simulink model "OSWEC_RO"  (R2023b)
settings: Solver=ode4  StartTime=0  StopTime=300  FixedStep=0.01  MaxStep=0.01  RelTol=1e-3  AbsTol=1e-3  EnableMultiTasking=on
values from neighbouring files (symbols this model uses):
  inertiaBlock = 1e-3    (= 0.001)    [wecSimInputFile.m]
  simu = simulationClass()    [wecSimInputFile.m]
undefined symbols (not defined in the file or in its folder): body, constraint, pto
libraries: fl_lib x17, nesl_utility x11, sh_lib x10, WECSim_Lib_Constraints x4, WECSim_Lib_Body_Elements x2, WECSim_Lib_Frames x1, sm_lib x1, fl_ps_legacy_lib x1, WECSim_Lib_PTOs x1
settings Model: Creator=mlawson  LastModifiedBy=jtgrasb
settings SolverCC: AutoScaleAbsTol=off  ZeroCrossControl=DisableAll  AlgebraicLoopSolver=TrustRegion  AutoInsertRateTranBlk=on
settings DataIOCC: SaveFormat=Array  SaveOutput=off  SaveTime=off  ReturnWorkspaceOutputs=off
settings OptimizationCC: LifeSpan=inf  SimCompilerOptimization=on
settings DebuggingCC: MergeDetectMultiDrivingBlocksExec=none  SolverPrmCheckMsg=warning  UnconnectedInputMsg=warning  UnconnectedOutputMsg=warning  UnconnectedLineMsg=warning  AllowSymbolicDim=off  StateNameClashWarn=warning  SFUnexpectedBacktrackingDiag=warning  SFNoUnconditionalDefaultTransitionDiag=warning  SFExecutionAtInitializationDiag=none  ArithmeticOperatorsInVariantConditions=warning
settings HardwareCC: ProdBitPerPointer=32  ProdBitPerSizeT=32  ProdBitPerPtrDiffT=32  ProdLargestAtomicFloat=None  ProdIntDivRoundTo=Undefined  ProdEndianess=Unspecified  ProdWordSize=32  ProdHWDeviceType=32-bit Generic
settings ModelReferenceCC: EnableRefExpFcnMdlSchedulingChecks=on  PropagateSignalLabelsOutOfModel=off
settings SFSimCC: SimUseLocalCustomCode=off  CustomCodeUndefinedFunction=UseInterfaceOnly
settings RTWCC: RTWUseLocalCustomCode=off  DLArmComputeVersion=19.05
settings CodeAppCC: StateflowObjectComments=on
settings GRTTargetCC: TargetLangStandard=C89/C90 (ANSI)
settings ConfigComp: CovMetricSettings=dw  CovSaveCumulativeToWorkspaceVar=on  CovSaveSingleToWorkspaceVar=on  CovExternalEMLEnable=off  CovSFcnEnable=off
settings SimscapeCC: SimscapeNormalizeSystem=off  SimscapeLogType=all  SimscapeLogLimitData=off  SimscapeLogDataHistory=100000
settings ConfigurationSet: Description=SimMechanics 2G
settings ExplorerConfigSet: SimMechanicsOpenEditorOnUpdate=off  InternalSimMechanicsExplorerSettings="<ExplorerConfiguration><canonicalview>default</canonicalview><TilePanel><TileInfo><Tiles Columns=\"1\" Count=\"1\" Rows=\"1\"><Column Left=\"2\" Weight=\"1\"/><Column Left=\"1335\"/><Row Top=\"2\" Weight=\"1\"/><Row Top=\"911\"/><Tile Height=\"1\" Width=\"1\" X=\"0\" Y=\"0\"/></Tiles></TileInfo><SceneInfo><SceneViewer><BGColor><R>0.60000002384185791</R><G>0.60000002384185791</G><B>0.60000002384185791</B></BGColor><Camera><Position><X>365.37645888990272</X><Y>-369.82486814446582</Y><Z>359.64809521743916</Z></Position><Center><X>-6.7351450971904585</X><Y>2.2867358426280204</Y><Z>-12.463508769654169</Z></Center><Up><X>-0.40824829046386307</X><Y>0.40824829046386307</Y><Z>0.81649658092772615</Z></Up><Left>-57.820127362122818</Left><Right>57.820127362122818</Right><Bottom>-38.308817187253304</Bottom><Top>38.308817187253304</Top></Camera></SceneViewer></SceneInfo></TilePanel></ExplorerConfiguration>"

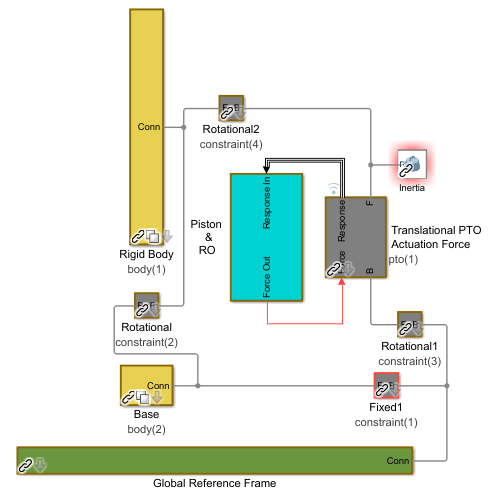
[thumbnail: Simulink's stored preview of the top-level diagram]
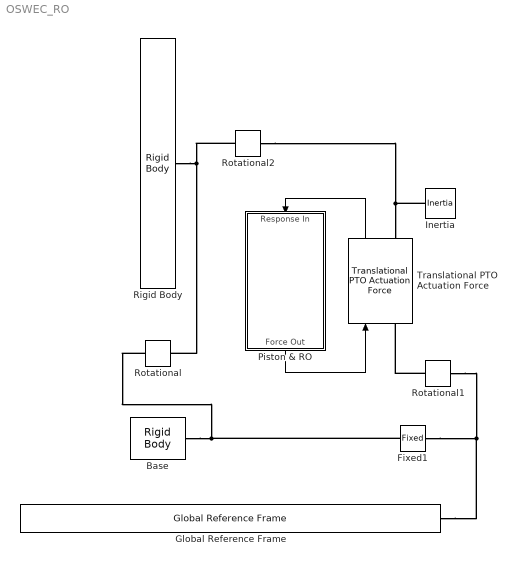
== system OSWEC_RO ==
  Base : WECSim_Lib_Body_Elements/Rigid Body  body=body(2)
  Fixed1 : WECSim_Lib_Constraints/Fixed  constraint=constraint(1)
      settings: AttributesFormatString=%<constraint>
  Global Reference Frame : WECSim_Lib_Frames/Global Reference Frame  waves=waves  simu=simu
  Inertia : sm_lib/Body Elements/Inertia  InertiaType=PointMass  Mass=inertiaBlock  MassUnits=kg  CenterOfMass=[0 0 0]  CenterOfMassUnits=m  MomentsOfInertia=[1 1 1]  MomentsOfInertiaUnits=kg*m^2  ProductsOfInertia=[1 1 1]  ProductsOfInertiaUnits=kg*m^2  GraphicType=Marker  MarkerShape=Inertia  MarkerSize=20  GraphicVisPropType=SimpleVisualProperties  GraphicDiffuseColor=[0.5 0.5 0.5]  GraphicSpecularColor=[0.5 0.5 0.5 1.0]  GraphicAmbientColor=[0.15 0.15 0.15 1.0]  GraphicEmissiveColor=[0.0 0.0 0.0 1.0]  GraphicShininess=75  GraphicOpacity=1.0
  "Piston & RO   " : Subsystem
  Rigid Body : WECSim_Lib_Body_Elements/Rigid Body  body=body(1)
  Rotational : WECSim_Lib_Constraints/Rotational  constraint=constraint(2)
      settings: AttributesFormatString=%<constraint>
  Rotational1 : WECSim_Lib_Constraints/Rotational  constraint=constraint(3)
      settings: AttributesFormatString=%<constraint>
  Rotational2 : WECSim_Lib_Constraints/Rotational  constraint=constraint(4)
      settings: AttributesFormatString=%<constraint>
  Translational PTO Actuation Force : WECSim_Lib_PTOs/Translational PTO Actuation Force  pto=pto(1)
      settings: AttributesFormatString=%<pto>
  wires:
  "Piston & RO   "/1(Force Out) -> Translational PTO Actuation Force/1
  Translational PTO Actuation Force/1 -> "Piston & RO   "/1(Response In)
  connections:
  Fixed1/LConn1 -- Global Reference Frame/RConn1 -- Rotational1/LConn1
  Fixed1/RConn1 -- Rotational/LConn1 -- Base/RConn1
  Rotational2/RConn1 -- Rigid Body/RConn1 -- Rotational/RConn1
  Rotational1/RConn1 -- Translational PTO Actuation Force/LConn1
  Rotational2/LConn1 -- Inertia/RConn1 -- Translational PTO Actuation Force/RConn1

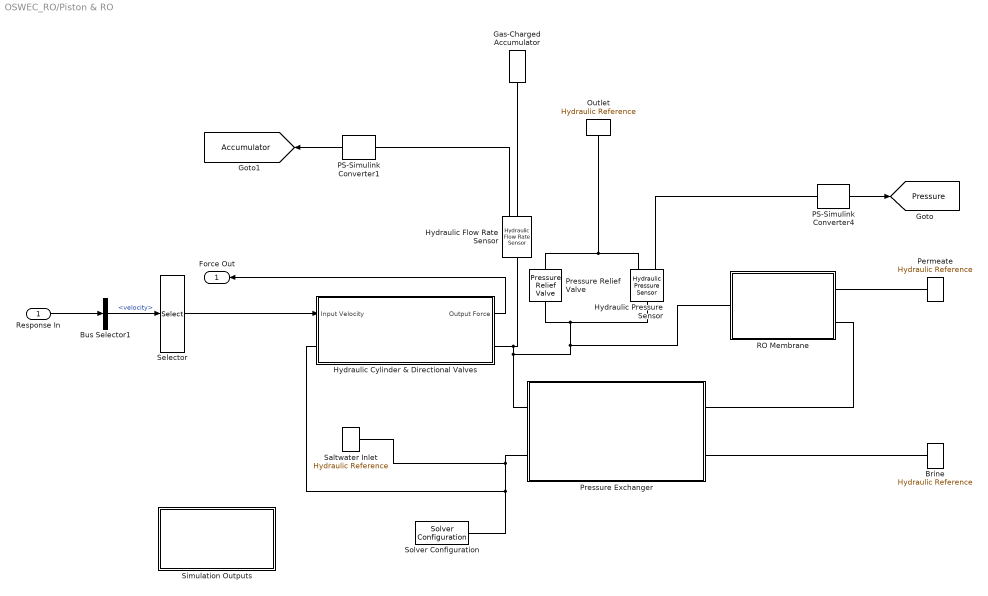
== system OSWEC_RO/Piston & RO    ==
  Response In : Inport
  "Brine " : fl_lib/Hydraulic/Hydraulic Elements/Hydraulic Reference
  Bus Selector1 : BusSelector  OutputSignals=velocity
  Gas-Charged Accumulator : sh_lib/Accumulators/Gas-Charged Accumulator  capacity=4 m^3  dead_volume=4e-5 m^3  pr_preload=30e5 Pa  k_sh=1.4  stiff_coeff=1e7 Pa/m^3  penetr_coeff=1e7 s*Pa/m^6  flow_rate_specify=off  flow_rate_priority=None  flow_rate=0 m^3/s  flow_rate_nominal_specify=off  flow_rate_nominal_unit=m^3/s  flow_rate_nominal_value=1  liquid_volume_specify=on  liquid_volume_priority=High  liquid_volume=0 m^3  liquid_volume_nominal_specify=off  liquid_volume_nominal_unit=m^3  liquid_volume_nominal_value=1  liquid_pressure_specify=off  liquid_pressure_priority=None  liquid_pressure=1.01325e+5 Pa  liquid_pressure_nominal_specify=off  liquid_pressure_nominal_unit=Pa  liquid_pressure_nominal_value=1
      settings: InternalSimscapePortConfiguration="{\"Bottom\":[],\"Left\":[],\"Right\":[{\"id\":\"A\",\"label\":\"A\",\"type\":\"foundation.hydraulic.hydraulic\"}],\"Top\":[]}"
  Hydraulic Flow Rate Sensor : fl_lib/Hydraulic/Hydraulic Sensors/Hydraulic Flow Rate Sensor
  Hydraulic Cylinder & Directional Valves : Subsystem
      mask Display: image('Images/HydraulicCylinder.png');
  Hydraulic Pressure Sensor : fl_lib/Hydraulic/Hydraulic Sensors/Hydraulic Pressure Sensor
  Outlet : fl_lib/Hydraulic/Hydraulic Elements/Hydraulic Reference
  PS-Simulink Converter1 : nesl_utility/PS-Simulink Converter  PhysicalDomain=network_engine_domain  SubClassName=ps_output  LeftPortType=input  RightPortType=output  PseudoPeriodic=off  Frequencies=[]  VectorFormat=1-D array  Unit=1  AffineConversion=off
  PS-Simulink Converter4 : nesl_utility/PS-Simulink Converter  PhysicalDomain=network_engine_domain  SubClassName=ps_output  LeftPortType=input  RightPortType=output  PseudoPeriodic=off  Frequencies=[]  VectorFormat=1-D array  Unit=1  AffineConversion=off
  Permeate : fl_lib/Hydraulic/Hydraulic Elements/Hydraulic Reference
  Pressure Relief Valve : sh_lib/Valves/Pressure Control Valves/Pressure Relief Valve  valve_area_spec=1  p_diff_TLU=[30.15e5 : 15e3 : 31.35e5] Pa  area_TLU=[1 : 1 : 9] .* 1e-5 m^2  area_max=2.67e-2 m^2  pres_set=56e5 Pa  reg_range=1e5 Pa  C_d=0.7  A_leak=1e-12 m^2  lam_spec=1  B_lam=0.999  Re_cr=12  dynamic=1  tau=0.1 s  area_init=1e-12 m^2
      settings: InternalSimscapePortConfiguration="{\"Bottom\":[],\"Left\":[{\"id\":\"A\",\"label\":\"A\",\"type\":\"foundation.hydraulic.hydraulic\"}],\"Right\":[{\"id\":\"B\",\"label\":\"B\",\"type\":\"foundation.hydraulic.hydraulic\"}],\"Top\":[]}"
  Pressure Exchanger : Subsystem
      mask Display: image('Images/PressureExchanger.png');
  RO Membrane : Subsystem
      mask Display: image('Images/ReverseOsmosisMembrane.jpg');
  Saltwater Inlet : fl_lib/Hydraulic/Hydraulic Elements/Hydraulic Reference
  Selector : Selector  InputPortWidth=6  IndexOptions=Index vector (dialog)  Indices=3  OutputSizes=1
  Simulation Outputs : Subsystem
  Solver Configuration : nesl_utility/Solver Configuration  PhysicalDomain=network_engine_domain  SubClassName=solver  LeftPortType=input  RightPortType=generic  Tones=[]  Harmonics=[]  SimulateNoise=off  Profile=off  UseLocalSampling=off  EnableSwitchedLinearOptims=on  FrequencyDomain=off  UseCCode=off  RelTol=0.001  AbsTol=1e-06  MinStep=1e-09  ToWorkspace=off  RevertToSquareIcSolve=off  NumHomotopyIterations=100  PhasorMode=off  PhasorModeNumHarmonics=1  ConsistencySolver=NEWTON_FTOL  IndexReductionMethod=DerivativeReplacement  DoDC=on  ResidualTolerance=1e-09  ConsistencyTolSource=GLOBAL  ConsistencyAbsTol=0.001  ConsistencyRelTol=0.001  ConsistencyTolFactor=0.001  UseLocalSolver=on  LocalSolverChoice=NE_BACKWARD_EULER_ADVANCER  ResolveIndetEquations=on  FunctionEvalNumThread=1  LocalSolverSampleTime=simu.dt  DoFixedCost=on  MaxNonlinIter=3  MaxModeIter=2  ComputeImpulses=off  ImpulseIterations=2  LinearAlgebra=Sparse  LinearAlgebraNumThread=0  EquationFormulation=NE_TIME_EF  DelaysMemoryBudget=1024  AutomaticFiltering=on  FilteringTimeConstant=0.001  PartitionStorageMethod=AS_NEEDED  PartitionMemoryBudget=1024  PartitionMethod=FAST  MultibodyUseLocalSolver=off  MultibodyLocalSolverChoice=ODE1  MultibodyLocalSolverSampleTime=0.001
  Force Out : Outport  VectorParamsAs1DForOutWhenUnconnected=off
  tag scope: Accumulator=global, Pressure=global
  wires:
  Hydraulic Cylinder & Directional Valves/1(Output Force) -> Force Out/1
  PS-Simulink Converter4/1 -> [Pressure]
  PS-Simulink Converter1/1 -> [Accumulator]
  Response In/1 -> Bus Selector1/1
  Bus Selector1/1 -> Selector/1  "<velocity>"
  Selector/1 -> Hydraulic Cylinder & Directional Valves/1(Input Velocity)
  connections:
  Hydraulic Cylinder & Directional Valves/LConn1 -- Pressure Exchanger/LConn2 -- Saltwater Inlet/LConn1 -- Solver Configuration/RConn1
  Outlet/LConn1 -- Hydraulic Pressure Sensor/RConn1 -- Pressure Relief Valve/RConn1
  Permeate/LConn1 -- RO Membrane/RConn1
  PS-Simulink Converter4/LConn1 -- Hydraulic Pressure Sensor/RConn2
  RO Membrane/RConn2 -- Pressure Exchanger/RConn1
  "Brine "/LConn1 -- Pressure Exchanger/RConn2
  Hydraulic Flow Rate Sensor/RConn1 -- PS-Simulink Converter1/LConn1
  Hydraulic Cylinder & Directional Valves/RConn1 -- Hydraulic Flow Rate Sensor/LConn1 -- Pressure Exchanger/LConn1 -- Hydraulic Pressure Sensor/LConn1 -- Pressure Relief Valve/LConn1 -- RO Membrane/LConn1
  Hydraulic Flow Rate Sensor/RConn2 -- Gas-Charged Accumulator/RConn1

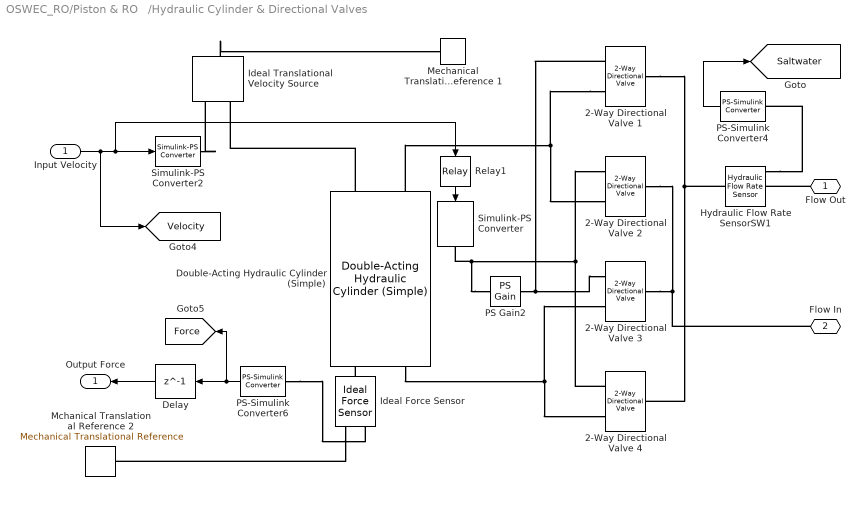
== system OSWEC_RO/Piston & RO   /Hydraulic Cylinder & Directional Valves ==
  Input Velocity : Inport
  2-Way Directional Valve {1..4} (4 alike) : sh_lib/Valves/Directional Valves/2-Way Directional Valve  mdl_type=1  area_max=5e-2 m^2  opening_max=1 m  opening_tab=[-0.002, 0.0, 0.002, 0.005, 0.015] m  area_tab=[1.0e-9, 2.0352e-7, 4.0736e-5, 0.00011438, 0.00034356] m^2  pressure_tab=[-10000000.0, -5000000.0, -2000000.0, 2000000.0, 5000000.0, 10000000.0] Pa  flow_rate_tab=[-1.0e-7, -7.0711e-8, -4.4721e-8, 4.4721e-8, 7.0711e-8, 1.0e-7; -2.0352e-5, -1.4391e-5, -9.1017e-6, 9.1017e-6, 1.4391e-5, 2.0352e-5; -0.0040736, -0.0028805, -0.0018218, 0.0018218, 0.0028805, 0.0040736; -0.011438, -0.0080879, -0.0051152, 0.0051152, 0.0080879, 0.011438; -0.034356, -0.024293, -0.015364, 0.015364, 0.024293, 0.034356] m^3/s  interp_method=1  extrap_method=1  C_d=0.7  x_0=0 m  A_leak=1e-8 m^2  lam_spec=1  B_lam=0.999  Re_cr=12
      settings: InternalSimscapePortConfiguration="{\"Bottom\":[],\"Left\":[{\"id\":\"S\",\"label\":\"S\",\"type\":\"input\"},{\"id\":\"A\",\"label\":\"A\",\"type\":\"foundation.hydraulic.hydraulic\"}],\"Right\":[{\"id\":\"B\",\"label\":\"B\",\"type\":\"foundation.hydraulic.hydraulic\"}],\"Top\":[]}"
  Delay : Delay  DelayLength=1  InitialCondition=0
  Double-Acting Hydraulic Cylinder (Simple) : sh_lib/Hydraulic Cylinders/Double-Acting Hydraulic Cylinder (Simple)  area_A=0.26 m^2  area_B=0.26 m^2  stroke=12 m  init_pos=6 m  penetr_coeff=1e12 s*N/m^2  or=1
      settings: InternalSimscapePortConfiguration="{\"Bottom\":[],\"Left\":[{\"id\":\"C\",\"label\":\"C\",\"type\":\"foundation.mechanical.translational.translational\"},{\"id\":\"A\",\"label\":\"A\",\"type\":\"foundation.hydraulic.hydraulic\"}],\"Right\":[{\"id\":\"R\",\"label\":\"R\",\"type\":\"foundation.mechanical.translational.translational\"},{\"id\":\"B\",\"label\":\"B\",\"type\":\"foundation.hydraulic.hydraulic\"}],\"Top\":[]}"
  Hydraulic Flow Rate SensorSW1 : fl_lib/Hydraulic/Hydraulic Sensors/Hydraulic Flow Rate Sensor
  Ideal Force Sensor : fl_lib/Mechanical/Mechanical Sensors/Ideal Force Sensor
  Ideal Translational Velocity Source : fl_lib/Mechanical/Mechanical Sources/Ideal Translational Velocity Source
  Mchanical Translational Reference 2 : fl_lib/Mechanical/Translational Elements/Mechanical Translational Reference
  Mechanical Translational Reference 1 : fl_lib/Mechanical/Translational Elements/Mechanical Translational Reference
  PS Gain2 : fl_ps_legacy_lib/Legacy Physical Signals/Functions/PS Gain  gain=-1
  PS-Simulink Converter4 : nesl_utility/PS-Simulink Converter  PhysicalDomain=network_engine_domain  SubClassName=ps_output  LeftPortType=input  RightPortType=output  PseudoPeriodic=off  Frequencies=[]  VectorFormat=1-D array  Unit=1  AffineConversion=off
  PS-Simulink Converter6 : nesl_utility/PS-Simulink Converter  PhysicalDomain=network_engine_domain  SubClassName=ps_output  LeftPortType=input  RightPortType=output  PseudoPeriodic=off  Frequencies=[]  VectorFormat=1-D array  Unit=1  AffineConversion=off
  Relay1 : Relay  OnSwitchValue=0  OffSwitchValue=0  OffOutputValue=-1  ZeroCross=off
  Simulink-PS Converter : nesl_utility/Simulink-PS Converter  PhysicalDomain=network_engine_domain  SubClassName=ps_input  LeftPortType=input  RightPortType=output  PseudoPeriodic=off  Frequencies=[]  NoiseDistribution=none  NoiseParameters=[]  Unit=1  AffineConversion=off  FilteringAndDerivatives=provide  SimscapeFilterOrder=2  InputFilterTimeConstant=0.01  UdotUserProvided=0
  Simulink-PS Converter2 : nesl_utility/Simulink-PS Converter  PhysicalDomain=network_engine_domain  SubClassName=ps_input  LeftPortType=input  RightPortType=output  PseudoPeriodic=off  Frequencies=[]  NoiseDistribution=none  NoiseParameters=[]  Unit=1  AffineConversion=off  FilteringAndDerivatives=provide  SimscapeFilterOrder=1  InputFilterTimeConstant=0.01  UdotUserProvided=0
  Flow Out : PMIOPort  Side=Right
  Flow In : PMIOPort  Port=2  Side=Left
  Output Force : Outport  VectorParamsAs1DForOutWhenUnconnected=off
  tag scope: Force=global, Saltwater=global, Velocity=global
  wires:
  Relay1/1 -> Simulink-PS Converter/1
  PS-Simulink Converter6/1 -> Delay/1, [Force]
  Input Velocity/1 -> [Velocity], Relay1/1, Simulink-PS Converter2/1
  Delay/1 -> Output Force/1
  PS-Simulink Converter4/1 -> [Saltwater]
  connections:
  2-Way Directional Valve 1/LConn2 -- Double-Acting Hydraulic Cylinder (Simple)/RConn2 -- 2-Way Directional Valve 2/LConn2
  2-Way Directional Valve 1/RConn1 -- Hydraulic Flow Rate SensorSW1/LConn1 -- 2-Way Directional Valve 4/RConn1
  2-Way Directional Valve 3/RConn1 -- Flow In/RConn1 -- 2-Way Directional Valve 2/RConn1
  2-Way Directional Valve 3/LConn1 -- 2-Way Directional Valve 1/LConn1 -- PS Gain2/RConn1
  Double-Acting Hydraulic Cylinder (Simple)/LConn2 -- 2-Way Directional Valve 3/LConn2 -- 2-Way Directional Valve 4/LConn2
  PS Gain2/LConn1 -- Simulink-PS Converter/RConn1 -- 2-Way Directional Valve 4/LConn1 -- 2-Way Directional Valve 2/LConn1
  Ideal Translational Velocity Source/LConn1 -- Mechanical Translational Reference 1/LConn1
  Simulink-PS Converter2/RConn1 -- Ideal Translational Velocity Source/RConn1
  PS-Simulink Converter6/LConn1 -- Ideal Force Sensor/RConn2
  Double-Acting Hydraulic Cylinder (Simple)/RConn1 -- Ideal Translational Velocity Source/RConn2
  Hydraulic Flow Rate SensorSW1/RConn1 -- PS-Simulink Converter4/LConn1
  Flow Out/RConn1 -- Hydraulic Flow Rate SensorSW1/RConn2
  Ideal Force Sensor/LConn1 -- Double-Acting Hydraulic Cylinder (Simple)/LConn1
  Ideal Force Sensor/RConn1 -- Mchanical Translational Reference 2/LConn1

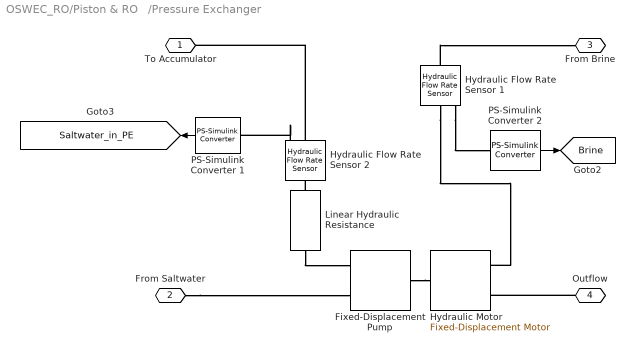
== system OSWEC_RO/Piston & RO   /Pressure Exchanger ==
  Fixed-Displacement Pump : sh_lib/Pumps and Motors/Fixed-Displacement Pump  D=(5e-6)*0.95 m^3/rad  loss_spec=1  w_nominal=188 rad/s  pr_nominal=100e5 Pa  visc_nominal=18 cSt  dens_nominal=900 kg/m^3  efficiency_vol=1  no_load_torque=0 N*m  torque_pressure_coeff=1*(5e-6)*((1)/(1)-1 ) N*m/Pa  p_diff_eff_TLU=[100000.0, 1000000.0, 2000000.0] Pa  omega_eff_TLU=[25.0, 50.0, 100.0, 200.0, 300.0, 400.0] rad/s  vol_eff_TLU=[0.816, 0.908, 0.954, 0.977, 0.981, 0.984; 0.325, 0.663, 0.831, 0.916, 0.925, 0.946; 0.137, 0.568, 0.78, 0.892, 0.893, 0.91]  mech_eff_TLU=[0.996, 0.996, 0.996, 0.996, 0.996, 0.996; 0.988, 0.989, 0.989, 0.989, 0.989, 0.99; 0.981, 0.981, 0.982, 0.982, 0.983, 0.984]  p_diff_loss_TLU=[100000.0, 1000000.0, 2000000.0] Pa  omega_loss_TLU=[25.0, 50.0, 100.0, 200.0, 300.0, 400.0] rad/s  vol_loss_TLU=[0.023, 0.023, 0.023, 0.023, 0.0285, 0.032; 0.0844, 0.0842, 0.0845, 0.084, 0.1125, 0.108; 0.1079, 0.108, 0.11, 0.108, 0.1605, 0.18] * 1e-3 m^3/s  mech_loss_TLU=[0.002, 0.002, 0.002, 0.002, 0.002, 0.002; 0.0607, 0.0556, 0.0556, 0.0556, 0.0556, 0.0505; 0.1937, 0.1937, 0.1833, 0.1833, 0.1729, 0.1626] N*m  pressure_threshold=1e5 Pa  omega_threshold=10 rad/s  quadrant_check=0  pressure_check=0  min_valid_pressure=0 Pa  vol_eff_min=1e-3  vol_eff_max=1  mech_eff_min=1e-3  mech_eff_max=1
      settings: InternalSimscapePortConfiguration="{\"Bottom\":[],\"Left\":[{\"id\":\"S\",\"label\":\"S\",\"type\":\"foundation.mechanical.rotational.rotational\"}],\"Right\":[{\"id\":\"P\",\"label\":\"P\",\"type\":\"foundation.hydraulic.hydraulic\"},{\"id\":\"T\",\"label\":\"T\",\"type\":\"foundation.hydraulic.hydraulic\"}],\"Top\":[]}"
  Hydraulic Motor : sh_lib/Pumps and Motors/Fixed-Displacement Motor  D=5e-6 m^3/rad  loss_spec=1  w_nominal=188 rad/s  pr_nominal=100e5 Pa  visc_nominal=18 cSt  dens_nominal=900 kg/m^3  efficiency_vol=1  no_load_torque=0 N*m  torque_pressure_coeff=1*(5e-6)*( 1-(1)/(1)) N*m/Pa  p_diff_eff_TLU=[100000.0, 1000000.0, 2000000.0] Pa  omega_eff_TLU=[25.0, 50.0, 100.0, 200.0, 300.0, 400.0] rad/s  vol_eff_TLU=[0.816, 0.908, 0.954, 0.977, 0.981, 0.984; 0.325, 0.663, 0.831, 0.916, 0.925, 0.946; 0.137, 0.568, 0.78, 0.892, 0.893, 0.91]  mech_eff_TLU=[0.996, 0.996, 0.996, 0.996, 0.996, 0.996; 0.988, 0.989, 0.989, 0.989, 0.989, 0.99; 0.981, 0.981, 0.982, 0.982, 0.983, 0.984]  p_diff_loss_TLU=[100000.0, 1000000.0, 2000000.0] Pa  omega_loss_TLU=[25.0, 50.0, 100.0, 200.0, 300.0, 400.0] rad/s  vol_loss_TLU=[0.0282, 0.0253, 0.0241, 0.0235, 0.0291, 0.0325; 0.2596, 0.1271, 0.1017, 0.0917, 0.1216, 0.1142; 0.7874, 0.1901, 0.141, 0.1211, 0.1797, 0.1978] * 1e-3 m^3/s  mech_loss_TLU=[0.002, 0.002, 0.002, 0.002, 0.002, 0.002; 0.06, 0.055, 0.055, 0.055, 0.055, 0.05; 0.19, 0.19, 0.18, 0.18, 0.17, 0.16] N*m  pressure_threshold=1e5 Pa  omega_threshold=10 rad/s  quadrant_check=0  pressure_check=0  min_valid_pressure=0 Pa  vol_eff_min=1e-3  vol_eff_max=1  mech_eff_min=1e-3  mech_eff_max=1
      settings: InternalSimscapePortConfiguration="{\"Bottom\":[],\"Left\":[{\"id\":\"A\",\"label\":\"A\",\"type\":\"foundation.hydraulic.hydraulic\"},{\"id\":\"B\",\"label\":\"B\",\"type\":\"foundation.hydraulic.hydraulic\"}],\"Right\":[{\"id\":\"S\",\"label\":\"S\",\"type\":\"foundation.mechanical.rotational.rotational\"}],\"Top\":[]}"
  Hydraulic Flow Rate Sensor 1 : fl_lib/Hydraulic/Hydraulic Sensors/Hydraulic Flow Rate Sensor
  Hydraulic Flow Rate Sensor 2 : fl_lib/Hydraulic/Hydraulic Sensors/Hydraulic Flow Rate Sensor
  Linear Hydraulic Resistance : fl_lib/Hydraulic/Hydraulic Elements/Linear Hydraulic Resistance  resistance=0.6023e8/22 Pa/(m^3/s)  q_specify=off  q_priority=None  q=0.001 m^3/s  q_nominal_specify=off  q_nominal_unit=m^3/s  q_nominal_value=1  p_specify=off  p_priority=None  p=0 Pa  p_nominal_specify=off  p_nominal_unit=Pa  p_nominal_value=1
      settings: InternalSimscapePortConfiguration="{\"Bottom\":[],\"Left\":[{\"id\":\"A\",\"label\":\"A\",\"type\":\"foundation.hydraulic.hydraulic\"}],\"Right\":[{\"id\":\"B\",\"label\":\"B\",\"type\":\"foundation.hydraulic.hydraulic\"}],\"Top\":[]}"
  PS-Simulink Converter 1 : nesl_utility/PS-Simulink Converter  PhysicalDomain=network_engine_domain  SubClassName=ps_output  LeftPortType=input  RightPortType=output  PseudoPeriodic=off  Frequencies=[]  VectorFormat=1-D array  Unit=1  AffineConversion=off
  PS-Simulink Converter 2 : nesl_utility/PS-Simulink Converter  PhysicalDomain=network_engine_domain  SubClassName=ps_output  LeftPortType=input  RightPortType=output  PseudoPeriodic=off  Frequencies=[]  VectorFormat=1-D array  Unit=1  AffineConversion=off
  To Accumulator : PMIOPort  Side=Left
  From Saltwater : PMIOPort  Port=2  Side=Left
  From Brine : PMIOPort  Port=3  Side=Right
  Outflow : PMIOPort  Port=4  Side=Right
  tag scope: Brine=global, Saltwater_in_PE=global
  wires:
  PS-Simulink Converter 2/1 -> [Brine]
  PS-Simulink Converter 1/1 -> [Saltwater_in_PE]
  connections:
  Fixed-Displacement Pump/LConn1 -- Hydraulic Motor/RConn1
  Hydraulic Flow Rate Sensor 1/RConn1 -- PS-Simulink Converter 2/LConn1
  Hydraulic Flow Rate Sensor 2/RConn1 -- PS-Simulink Converter 1/LConn1
  Linear Hydraulic Resistance/LConn1 -- Fixed-Displacement Pump/RConn1
  Hydraulic Flow Rate Sensor 1/RConn2 -- Hydraulic Motor/LConn1
  Linear Hydraulic Resistance/RConn1 -- Hydraulic Flow Rate Sensor 2/LConn1
  From Saltwater/RConn1 -- Fixed-Displacement Pump/RConn2
  Hydraulic Flow Rate Sensor 2/RConn2 -- To Accumulator/RConn1
  Hydraulic Flow Rate Sensor 1/LConn1 -- From Brine/RConn1
  Outflow/RConn1 -- Hydraulic Motor/LConn2

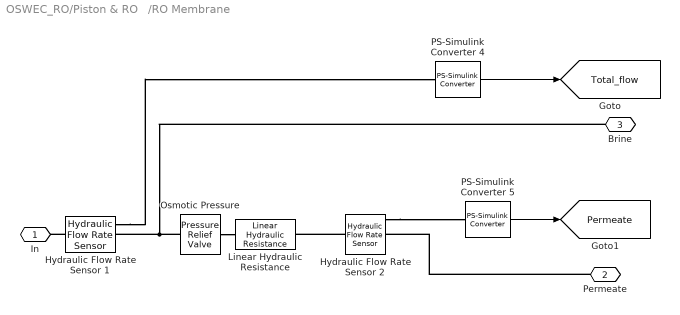
== system OSWEC_RO/Piston & RO   /RO Membrane ==
  Hydraulic Flow Rate Sensor 1 : fl_lib/Hydraulic/Hydraulic Sensors/Hydraulic Flow Rate Sensor
  Hydraulic Flow Rate Sensor 2 : fl_lib/Hydraulic/Hydraulic Sensors/Hydraulic Flow Rate Sensor
  Linear Hydraulic Resistance : fl_lib/Hydraulic/Hydraulic Elements/Linear Hydraulic Resistance  resistance=0.6023e8 Pa/(m^3/s)  q_specify=off  q_priority=None  q=0.001 m^3/s  q_nominal_specify=off  q_nominal_unit=m^3/s  q_nominal_value=1  p_specify=off  p_priority=None  p=0 Pa  p_nominal_specify=off  p_nominal_unit=Pa  p_nominal_value=1
      settings: InternalSimscapePortConfiguration="{\"Bottom\":[],\"Left\":[{\"id\":\"A\",\"label\":\"A\",\"type\":\"foundation.hydraulic.hydraulic\"}],\"Right\":[{\"id\":\"B\",\"label\":\"B\",\"type\":\"foundation.hydraulic.hydraulic\"}],\"Top\":[]}"
  Osmotic Pressure : sh_lib/Valves/Pressure Control Valves/Pressure Relief Valve  valve_area_spec=1  p_diff_TLU=[30.15e5 : 15e3 : 31.35e5] Pa  area_TLU=[1 : 1 : 9] .* 1e-5 m^2  area_max=3e-1 m^2  pres_set=30e5 Pa  reg_range=5e4 Pa  C_d=0.7  A_leak=1e-12 m^2  lam_spec=1  B_lam=0.999  Re_cr=12  dynamic=0  tau=0.1 s  area_init=1e-12 m^2
      settings: InternalSimscapePortConfiguration="{\"Bottom\":[],\"Left\":[{\"id\":\"A\",\"label\":\"A\",\"type\":\"foundation.hydraulic.hydraulic\"}],\"Right\":[{\"id\":\"B\",\"label\":\"B\",\"type\":\"foundation.hydraulic.hydraulic\"}],\"Top\":[]}"
  PS-Simulink Converter 4 : nesl_utility/PS-Simulink Converter  PhysicalDomain=network_engine_domain  SubClassName=ps_output  LeftPortType=input  RightPortType=output  PseudoPeriodic=off  Frequencies=[]  VectorFormat=1-D array  Unit=1  AffineConversion=off
  PS-Simulink Converter 5 : nesl_utility/PS-Simulink Converter  PhysicalDomain=network_engine_domain  SubClassName=ps_output  LeftPortType=input  RightPortType=output  PseudoPeriodic=off  Frequencies=[]  VectorFormat=1-D array  Unit=1  AffineConversion=off
  In : PMIOPort  Side=Left
  Permeate : PMIOPort  Port=2  Side=Right
  Brine : PMIOPort  Port=3  Side=Right
  tag scope: Permeate=global, Total_flow=global
  wires:
  PS-Simulink Converter 5/1 -> [Permeate]
  PS-Simulink Converter 4/1 -> [Total_flow]
  connections:
  Hydraulic Flow Rate Sensor 2/RConn1 -- PS-Simulink Converter 5/LConn1
  Hydraulic Flow Rate Sensor 1/RConn1 -- PS-Simulink Converter 4/LConn1
  Hydraulic Flow Rate Sensor 1/LConn1 -- In/RConn1
  Permeate/RConn1 -- Hydraulic Flow Rate Sensor 2/RConn2
  Hydraulic Flow Rate Sensor 2/LConn1 -- Linear Hydraulic Resistance/RConn1
  Osmotic Pressure/RConn1 -- Linear Hydraulic Resistance/LConn1
  Osmotic Pressure/LConn1 -- Brine/RConn1 -- Hydraulic Flow Rate Sensor 1/RConn2

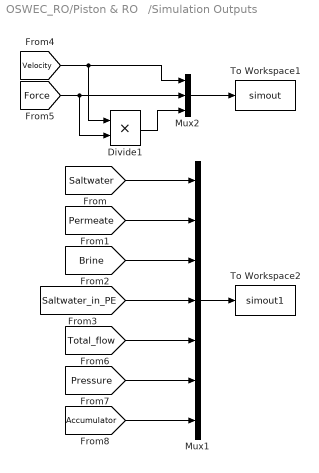
== system OSWEC_RO/Piston & RO   /Simulation Outputs ==
  Divide1 : Product  Inputs=**
  Mux1 : Mux  Inputs=7
  Mux2 : Mux  Inputs=3
  To Workspace1 : ToWorkspace  VariableName=simout  SaveFormat=Structure With Time  SampleTime=simu.dtOut
  To Workspace2 : ToWorkspace  VariableName=simout1  SaveFormat=Structure With Time  SampleTime=simu.dtOut
  wires:
  [Saltwater] -> Mux1/1
  [Permeate] -> Mux1/2
  Mux1/1 -> To Workspace2/1
  [Saltwater_in_PE] -> Mux1/4
  [Brine] -> Mux1/3
  [Force] -> Divide1/2, Mux2/2
  Divide1/1 -> Mux2/3
  [Velocity] -> Mux2/1, Divide1/1
  Mux2/1 -> To Workspace1/1
  [Total_flow] -> Mux1/5
  [Pressure] -> Mux1/6
  [Accumulator] -> Mux1/7
